simulink model "propellant_consuption_baseline"  (R2026a)
settings: Solver=VariableStepAuto
InitFcn:
  | model_dir = fileparts(get_param(bdroot, 'FileName'));
  | project_root = fileparts(fileparts(model_dir));
  | run(fullfile(project_root, 'scripts', 'matlab', 'setup_simulation.m'));
undefined symbols (not defined in the file): ch4_flow_kg_s, effective_exhaust_velocity_m_s, lox_flow_kg_s, ramp_duration_s, start_time_s, total_flow_kg_s
libraries: simulink x3
settings Model: Creator=giuse  LastModifiedBy=giuse

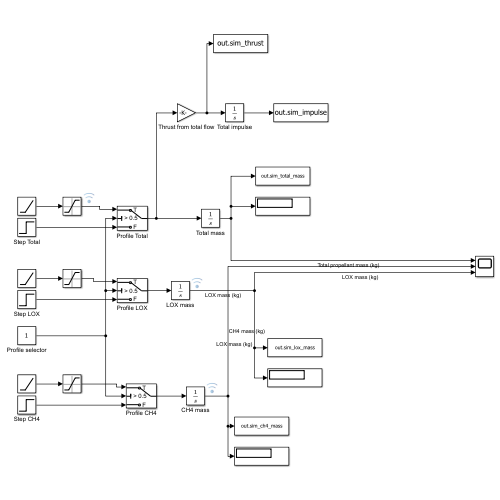
[thumbnail: Simulink's stored preview of the top-level diagram]
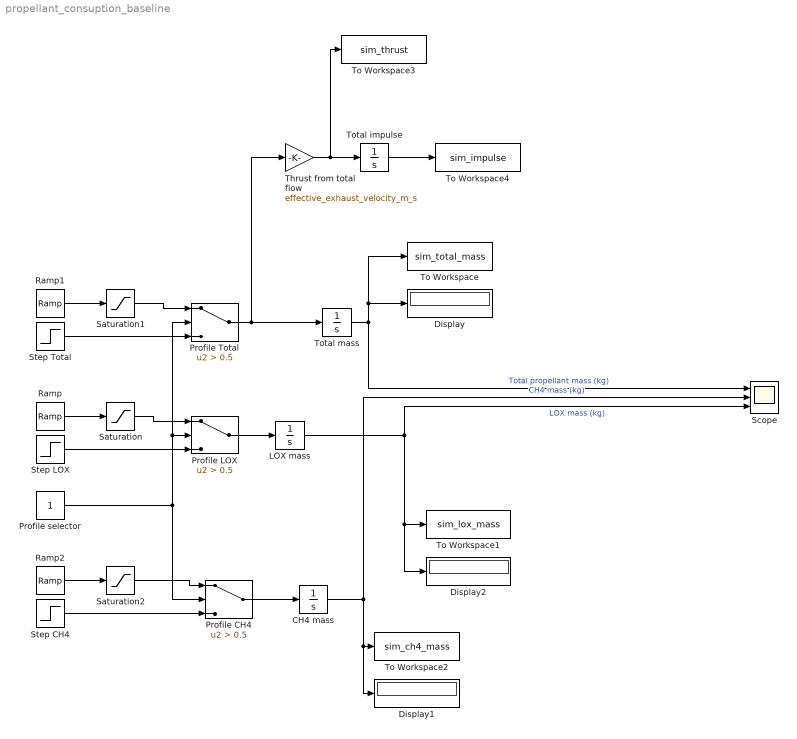
== system propellant_consuption_baseline ==
  CH4 mass : Integrator
  Display : Display
  Display1 : Display
  Display2 : Display
  LOX mass : Integrator
  Profile CH4 : Switch  Criteria=u2 > Threshold  Threshold=0.5  SaturateOnIntegerOverflow=off  InputSameDT=off
  Profile LOX : Switch  Criteria=u2 > Threshold  Threshold=0.5  SaturateOnIntegerOverflow=off  InputSameDT=off
  Profile Total : Switch  Criteria=u2 > Threshold  Threshold=0.5  SaturateOnIntegerOverflow=off  InputSameDT=off
  Profile selector : Constant
  Ramp : simulink/Sources/Ramp  slope=lox_flow_kg_s / ramp_duration_s  start=start_time_s  InitialOutput=0
  Ramp1 : simulink/Sources/Ramp  slope=total_flow_kg_s / ramp_duration_s  start=start_time_s  InitialOutput=0
  Ramp2 : simulink/Sources/Ramp  slope=ch4_flow_kg_s / ramp_duration_s  start=start_time_s  InitialOutput=0
  Saturation : Saturate  UpperLimit=lox_flow_kg_s  LowerLimit=0
  Saturation1 : Saturate  UpperLimit=total_flow_kg_s  LowerLimit=0
  Saturation2 : Saturate  UpperLimit=ch4_flow_kg_s  LowerLimit=0
  Scope : Scope  NumInputPorts=3
      settings: ActiveDisplayYMinimum=-2684.49671666137  ActiveDisplayYMaximum=5069.2508251765139
  Step CH4 : Step  Time=start_time_s  FinalValue=ch4_flow_kg_s  SampleTime=0
  Step LOX : Step  Time=start_time_s  FinalValue=lox_flow_kg_s  SampleTime=0
  Step Total : Step  Time=start_time_s  FinalValue=total_flow_kg_s  SampleTime=0
  Thrust from total flow : Gain  Gain=effective_exhaust_velocity_m_s
  To Workspace : ToWorkspace  VariableName=sim_total_mass  SaveFormat=Timeseries  SampleTime=-1
  To Workspace1 : ToWorkspace  VariableName=sim_lox_mass  SaveFormat=Timeseries  SampleTime=-1
  To Workspace2 : ToWorkspace  VariableName=sim_ch4_mass  SaveFormat=Timeseries  SampleTime=-1
  To Workspace3 : ToWorkspace  VariableName=sim_thrust  SaveFormat=Timeseries  SampleTime=-1
  To Workspace4 : ToWorkspace  VariableName=sim_impulse  SaveFormat=Timeseries  SampleTime=-1
  Total impulse : Integrator
  Total mass : Integrator
  wires:
  Total mass/1 -> To Workspace/1, Display/1, Scope/1  "Total propellant mass (kg)"
  LOX mass/1 -> Scope/3, Display2/1, To Workspace1/1  "LOX mass (kg)"
  CH4 mass/1 -> To Workspace2/1, Display1/1, Scope/2  "CH4 mass (kg)"
  Ramp/1 -> Saturation/1
  Ramp1/1 -> Saturation1/1
  Ramp2/1 -> Saturation2/1
  Profile selector/1 -> Profile CH4/2, Profile LOX/2, Profile Total/2
  Profile Total/1 -> Thrust from total flow/1, Total mass/1
  Saturation1/1 -> Profile Total/1
  Step Total/1 -> Profile Total/3
  Saturation/1 -> Profile LOX/1
  Step LOX/1 -> Profile LOX/3
  Saturation2/1 -> Profile CH4/1
  Step CH4/1 -> Profile CH4/3
  Profile LOX/1 -> LOX mass/1
  Profile CH4/1 -> CH4 mass/1
  Thrust from total flow/1 -> To Workspace3/1, Total impulse/1
  Total impulse/1 -> To Workspace4/1
